simulink model "temp_sensor_log"  (R2023b)
settings: Solver=VariableStepAuto  StartTime=0.0  StopTime=10.0  RelTol=1e-3
undefined symbols (not defined in the file or in its folder): a, a1, k, k1, reg, zz
settings Model: DataDictionary=main.sldd  Creator=Serjio  LastModifiedBy=Serjio

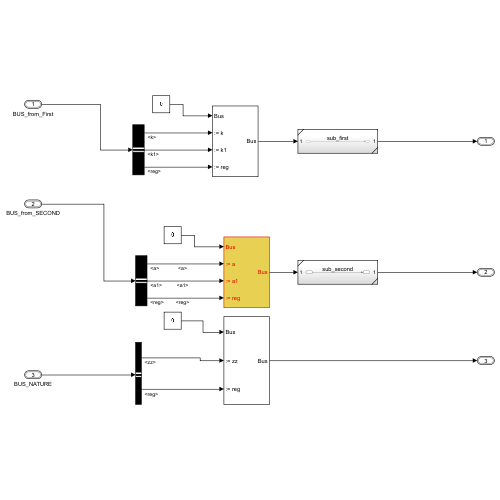
[thumbnail: Simulink's stored preview of the top-level diagram]
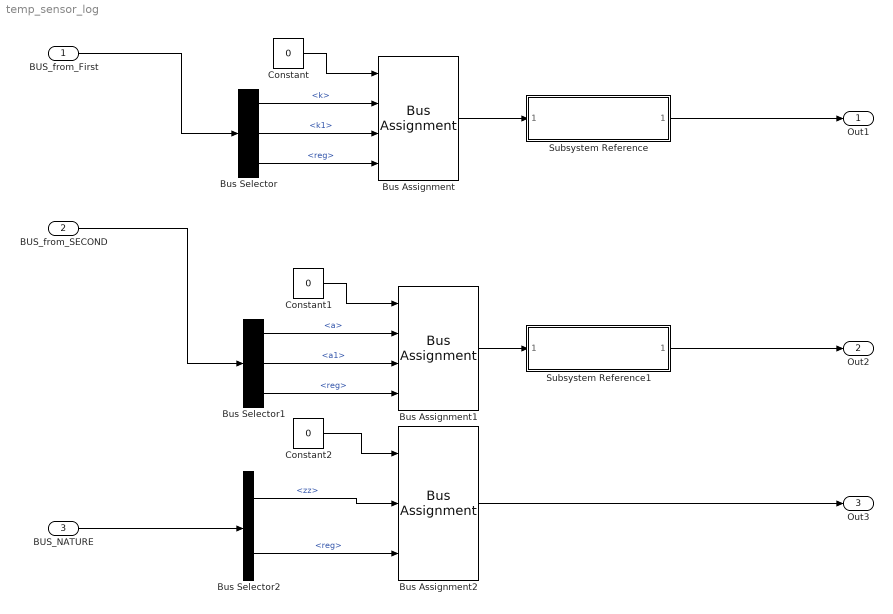
== system temp_sensor_log ==
  BUS_from_First : Inport  OutDataTypeStr=Bus: bs_mainF
  BUS_from_SECOND : Inport  Port=2  OutDataTypeStr=Bus: bs_second
  BUS_NATURE : Inport  Port=3  OutDataTypeStr=Bus: Bus_main
  Bus Assignment : BusAssignment  AssignedSignals=k,k1,reg
  Bus Assignment1 : BusAssignment  AssignedSignals=a,a1,reg
  Bus Assignment2 : BusAssignment  AssignedSignals=zz,reg
  Bus Selector : BusSelector  OutputSignals=k,k1,reg
  Bus Selector1 : BusSelector  OutputSignals=a,a1,reg
  Bus Selector2 : BusSelector  OutputSignals=zz,reg
  Constant : Constant  Value=0  OutDataTypeStr=Bus: bs_mainF
  Constant1 : Constant  Value=0  OutDataTypeStr=Bus: bs_second
  Constant2 : Constant  Value=0  OutDataTypeStr=Bus: Bus_main
  Subsystem Reference : Subsystem  ReferencedSubsystem=sub_first
      settings: PermitHierarchicalResolution=None
  Subsystem Reference1 : Subsystem  ReferencedSubsystem=sub_second
      settings: PermitHierarchicalResolution=None
  Out1 : Outport  OutDataTypeStr=Bus: bs_mainF
  Out2 : Outport  Port=2  OutDataTypeStr=Bus: bs_second
  Out3 : Outport  Port=3  OutDataTypeStr=Bus: Bus_main
  wires:
  BUS_from_First/1 -> Bus Selector/1
  BUS_from_SECOND/1 -> Bus Selector1/1
  Subsystem Reference/1 -> Out1/1
  Subsystem Reference1/1 -> Out2/1
  Bus Selector/1 -> Bus Assignment/2  "<k>"
  Bus Selector/2 -> Bus Assignment/3  "<k1>"
  Bus Selector/3 -> Bus Assignment/4  "<reg>"
  BUS_NATURE/1 -> Bus Selector2/1
  Bus Selector2/1 -> Bus Assignment2/2  "<zz>"
  Bus Selector2/2 -> Bus Assignment2/3  "<reg>"
  Constant/1 -> Bus Assignment/1
  Bus Assignment/1 -> Subsystem Reference/1
  Bus Assignment1/1 -> Subsystem Reference1/1
  Bus Selector1/3 -> Bus Assignment1/4  "<reg>"
  Constant1/1 -> Bus Assignment1/1
  Bus Selector1/2 -> Bus Assignment1/3  "<a1>"
  Bus Selector1/1 -> Bus Assignment1/2  "<a>"
  Bus Assignment2/1 -> Out3/1
  Constant2/1 -> Bus Assignment2/1
